simulink model "VirtualQuantumDotAgent"  (R2026a)
settings: Solver=FixedStepDiscrete  StartTime=0  StopTime=50e-9  FixedStep=1e-11
InitFcn:
  | qdEnsureWorkspace;
values from neighbouring files (symbols this model uses):
  QD_SAMPLE_TIME_S = 1.0e-11    (= 1e-11)    [initVirtualQuantumDotAgent.m]
  qdInput = qdDefaultInputs()    [initVirtualQuantumDotAgent.m]    (also in predictQDHybrid.m = defaults; predictQDWithError.m = defaults; qdDefaultInputs.m = struct(      'radius_nm', 3.0,      'temperature_K', 300.0, ; qdEnsureWorkspace.m = defaults)
undefined symbols (not defined in the file or in its folder): DiscIntNeverNeededParam
Description:
  | Virtual Quantum Dot Agent package model 1.2.0
settings Model: Creator=jyohtiprakash  LastModifiedBy=jyohtiprakash

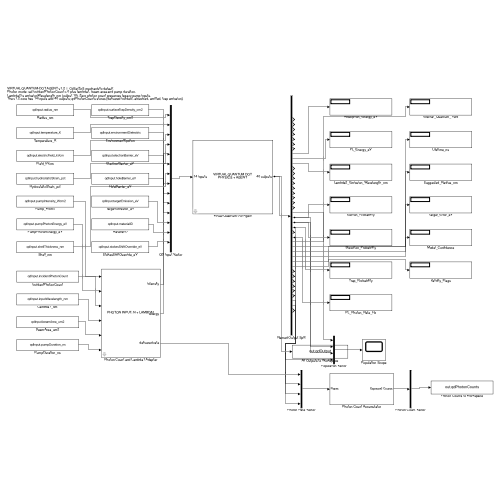
[thumbnail: Simulink's stored preview of the top-level diagram]
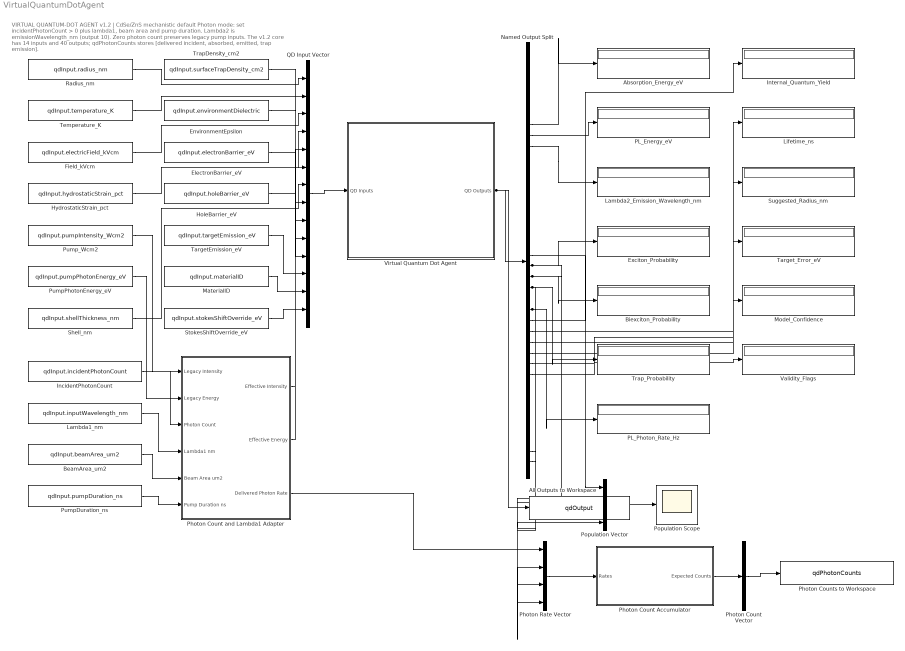
== system VirtualQuantumDotAgent ==
  note: VIRTUAL QUANTUM-DOT AGENT v1.2  |  CdSe/ZnS mechanistic default
      | Photon mode: set incidentPhotonCount > 0 plus lambda1, beam area and pump duration.
      | Lambda2 is emissionWavelength_nm (output 10). Zero photon count preserves legacy pump inputs.
      | The v1.2 core has 14 inputs and 40 outputs; qdPhotonCounts stores [delivered incident, absorbed, emitted, trap emission].
  Absorption_Energy_eV : Display
  All Outputs to Workspace : ToWorkspace  VariableName=qdOutput  SaveFormat=Structure With Time  SampleTime=-1
  BeamArea_um2 : Constant  Value=qdInput.beamArea_um2  SampleTime=QD_SAMPLE_TIME_S
  Biexciton_Probability : Display
  ElectronBarrier_eV : Constant  Value=qdInput.electronBarrier_eV  SampleTime=QD_SAMPLE_TIME_S
  EnvironmentEpsilon : Constant  Value=qdInput.environmentDielectric  SampleTime=QD_SAMPLE_TIME_S
  Exciton_Probability : Display
  Field_kVcm : Constant  Value=qdInput.electricField_kVcm  SampleTime=QD_SAMPLE_TIME_S
  HoleBarrier_eV : Constant  Value=qdInput.holeBarrier_eV  SampleTime=QD_SAMPLE_TIME_S
  HydrostaticStrain_pct : Constant  Value=qdInput.hydrostaticStrain_pct  SampleTime=QD_SAMPLE_TIME_S
  IncidentPhotonCount : Constant  Value=qdInput.incidentPhotonCount  SampleTime=QD_SAMPLE_TIME_S
  Internal_Quantum_Yield : Display
  Lambda1_nm : Constant  Value=qdInput.inputWavelength_nm  SampleTime=QD_SAMPLE_TIME_S
  Lambda2_Emission_Wavelength_nm : Display
  Lifetime_ns : Display
  MaterialID : Constant  Value=qdInput.materialID  SampleTime=QD_SAMPLE_TIME_S
  Model_Confidence : Display
  Named Output Split : Demux  Outputs=40
  PL_Energy_eV : Display
  PL_Photon_Rate_Hz : Display
  Photon Count Accumulator : Subsystem
  Photon Count Vector : Mux  Inputs=1
  Photon Count and Lambda1 Adapter : Subsystem
      mask help: Backward-compatible photon count and wavelength adapter for the 14-input quantum-dot core.
      mask Display:
      | disp('PHOTON INPUT: N + LAMBDA1');
      | port_label('output',1,'intensity');
      | port_label('output',2,'energy');
      | port_label('output',3,'delivered rate');
  Photon Counts to Workspace : ToWorkspace  VariableName=qdPhotonCounts  SaveFormat=Structure With Time  SampleTime=-1
  Photon Rate Vector : Mux
  Population Scope : Scope
  Population Vector : Mux
  PumpDuration_ns : Constant  Value=qdInput.pumpDuration_ns  SampleTime=QD_SAMPLE_TIME_S
  PumpPhotonEnergy_eV : Constant  Value=qdInput.pumpPhotonEnergy_eV  SampleTime=QD_SAMPLE_TIME_S
  Pump_Wcm2 : Constant  Value=qdInput.pumpIntensity_Wcm2  SampleTime=QD_SAMPLE_TIME_S
  QD Input Vector : Mux  Inputs=14
  Radius_nm : Constant  Value=qdInput.radius_nm  SampleTime=QD_SAMPLE_TIME_S
  Shell_nm : Constant  Value=qdInput.shellThickness_nm  SampleTime=QD_SAMPLE_TIME_S
  StokesShiftOverride_eV : Constant  Value=qdInput.stokesShiftOverride_eV  SampleTime=QD_SAMPLE_TIME_S
  Suggested_Radius_nm : Display
  TargetEmission_eV : Constant  Value=qdInput.targetEmission_eV  SampleTime=QD_SAMPLE_TIME_S
  Target_Error_eV : Display
  Temperature_K : Constant  Value=qdInput.temperature_K  SampleTime=QD_SAMPLE_TIME_S
  TrapDensity_cm2 : Constant  Value=qdInput.surfaceTrapDensity_cm2  SampleTime=QD_SAMPLE_TIME_S
  Trap_Probability : Display
  Validity_Flags : Display
  Virtual Quantum Dot Agent : Subsystem
      mask help: Effective-mass quantum-dot digital twin with population dynamics and inverse radius recommendation.
      mask Display:
      | disp('VIRTUAL QUANTUM DOT\nPHYSICS + AGENT');
      | port_label('input',1,'14 inputs');
      | port_label('output',1,'40 outputs');
  wires:
  Pump_Wcm2/1 -> Photon Count and Lambda1 Adapter/1(Legacy Intensity)
  PumpPhotonEnergy_eV/1 -> Photon Count and Lambda1 Adapter/2(Legacy Energy)
  IncidentPhotonCount/1 -> Photon Count and Lambda1 Adapter/3(Photon Count)
  Lambda1_nm/1 -> Photon Count and Lambda1 Adapter/4(Lambda1 nm)
  BeamArea_um2/1 -> Photon Count and Lambda1 Adapter/5(Beam Area um2)
  PumpDuration_ns/1 -> Photon Count and Lambda1 Adapter/6(Pump Duration ns)
  Radius_nm/1 -> QD Input Vector/1
  Temperature_K/1 -> QD Input Vector/2
  Field_kVcm/1 -> QD Input Vector/3
  HydrostaticStrain_pct/1 -> QD Input Vector/4
  Shell_nm/1 -> QD Input Vector/7
  TrapDensity_cm2/1 -> QD Input Vector/8
  EnvironmentEpsilon/1 -> QD Input Vector/9
  ElectronBarrier_eV/1 -> QD Input Vector/10
  HoleBarrier_eV/1 -> QD Input Vector/11
  TargetEmission_eV/1 -> QD Input Vector/12
  MaterialID/1 -> QD Input Vector/13
  StokesShiftOverride_eV/1 -> QD Input Vector/14
  Photon Count and Lambda1 Adapter/1(Effective Intensity) -> QD Input Vector/5
  Photon Count and Lambda1 Adapter/2(Effective Energy) -> QD Input Vector/6
  QD Input Vector/1 -> Virtual Quantum Dot Agent/1(QD Inputs)
  Virtual Quantum Dot Agent/1(QD Outputs) -> Named Output Split/1, All Outputs to Workspace/1
  Named Output Split/8 -> Absorption_Energy_eV/1
  Named Output Split/9 -> PL_Energy_eV/1
  Named Output Split/10 -> Lambda2_Emission_Wavelength_nm/1
  Named Output Split/21 -> Exciton_Probability/1, Population Vector/2
  Named Output Split/22 -> Biexciton_Probability/1, Population Vector/3
  Named Output Split/23 -> Trap_Probability/1, Population Vector/4
  Named Output Split/25 -> PL_Photon_Rate_Hz/1, Photon Rate Vector/3
  Named Output Split/26 -> Internal_Quantum_Yield/1
  Named Output Split/27 -> Lifetime_ns/1
  Named Output Split/28 -> Suggested_Radius_nm/1
  Named Output Split/29 -> Target_Error_eV/1
  Named Output Split/30 -> Model_Confidence/1
  Named Output Split/31 -> Validity_Flags/1
  Named Output Split/20 -> Population Vector/1
  Population Vector/1 -> Population Scope/1
  Photon Count and Lambda1 Adapter/3(Delivered Photon Rate) -> Photon Rate Vector/1
  Named Output Split/38 -> Photon Rate Vector/2
  Named Output Split/39 -> Photon Rate Vector/4
  Photon Rate Vector/1 -> Photon Count Accumulator/1(Rates)
  Photon Count Accumulator/1(Expected Counts) -> Photon Count Vector/1
  Photon Count Vector/1 -> Photon Counts to Workspace/1

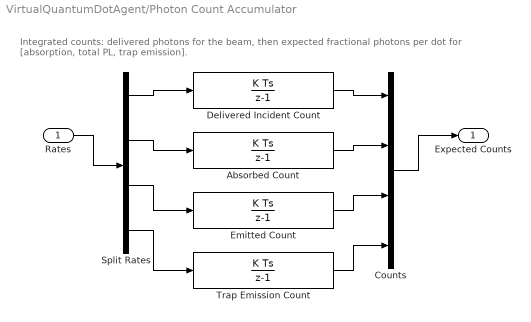
== system VirtualQuantumDotAgent/Photon Count Accumulator ==
  note: Integrated counts: delivered photons for the beam, then expected fractional photons per dot for [absorption, total PL, trap emission].
  Rates : Inport
  Absorbed Count : DiscreteIntegrator  gainval=1  SampleTime=QD_SAMPLE_TIME_S  ICPrevOutput=DiscIntNeverNeededParam  ICPrevScaledInput=DiscIntNeverNeededParam
  Counts : Mux
  Delivered Incident Count : DiscreteIntegrator  gainval=1  SampleTime=QD_SAMPLE_TIME_S  ICPrevOutput=DiscIntNeverNeededParam  ICPrevScaledInput=DiscIntNeverNeededParam
  Emitted Count : DiscreteIntegrator  gainval=1  SampleTime=QD_SAMPLE_TIME_S  ICPrevOutput=DiscIntNeverNeededParam  ICPrevScaledInput=DiscIntNeverNeededParam
  Split Rates : Demux
  Trap Emission Count : DiscreteIntegrator  gainval=1  SampleTime=QD_SAMPLE_TIME_S  ICPrevOutput=DiscIntNeverNeededParam  ICPrevScaledInput=DiscIntNeverNeededParam
  Expected Counts : Outport
  wires:
  Rates/1 -> Split Rates/1
  Split Rates/1 -> Delivered Incident Count/1
  Split Rates/2 -> Absorbed Count/1
  Split Rates/3 -> Emitted Count/1
  Split Rates/4 -> Trap Emission Count/1
  Delivered Incident Count/1 -> Counts/1
  Absorbed Count/1 -> Counts/2
  Emitted Count/1 -> Counts/3
  Trap Emission Count/1 -> Counts/4
  Counts/1 -> Expected Counts/1

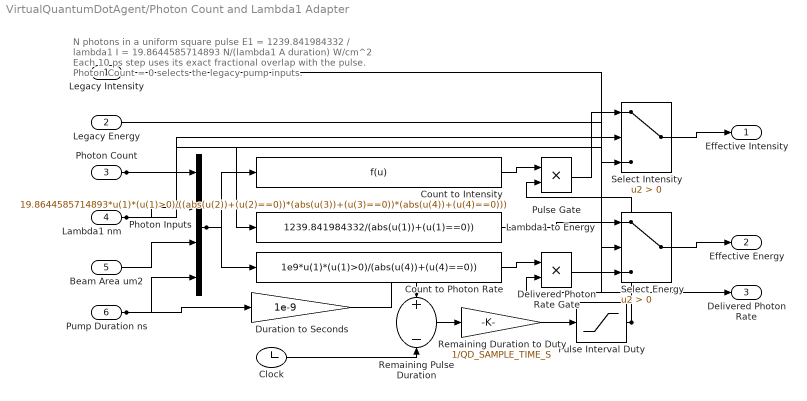
== system VirtualQuantumDotAgent/Photon Count and Lambda1 Adapter ==
  note: N photons in a uniform square pulse
      | E1 = 1239.841984332 / lambda1
      | I = 19.8644585714893 N/(lambda1 A duration) W/cm^2
      | Each 10 ps step uses its exact fractional overlap with the pulse.
      | Photon Count = 0 selects the legacy pump inputs.
  Legacy Intensity : Inport
  Legacy Energy : Inport  Port=2
  Photon Count : Inport  Port=3
  Lambda1 nm : Inport  Port=4
  Beam Area um2 : Inport  Port=5
  Pump Duration ns : Inport  Port=6
  Clock : Clock
  Count to Intensity : Fcn  Expr=19.8644585714893*u(1)*(u(1)>0)/((abs(u(2))+(u(2)==0))*(abs(u(3))+(u(3)==0))*(abs(u(4))+(u(4)==0)))
  Count to Photon Rate : Fcn  Expr=1e9*u(1)*(u(1)>0)/(abs(u(4))+(u(4)==0))
  Delivered Photon Rate Gate : Product  Inputs=**
  Duration to Seconds : Gain  Gain=1e-9
  Lambda1 to Energy : Fcn  Expr=1239.841984332/(abs(u(1))+(u(1)==0))
  Photon Inputs : Mux
  Pulse Gate : Product  Inputs=**
  Pulse Interval Duty : Saturate  UpperLimit=1  LowerLimit=0
  Remaining Duration to Duty : Gain  Gain=1/QD_SAMPLE_TIME_S
  Remaining Pulse Duration : Sum  Inputs=+-
  Select Energy : Switch  Criteria=u2 > Threshold  SaturateOnIntegerOverflow=off  InputSameDT=off
  Select Intensity : Switch  Criteria=u2 > Threshold  SaturateOnIntegerOverflow=off  InputSameDT=off
  Effective Intensity : Outport
  Effective Energy : Outport  Port=2
  Delivered Photon Rate : Outport  Port=3
  wires:
  Photon Count/1 -> Photon Inputs/1, Select Intensity/2, Select Energy/2
  Lambda1 nm/1 -> Photon Inputs/2, Lambda1 to Energy/1
  Beam Area um2/1 -> Photon Inputs/3
  Pump Duration ns/1 -> Photon Inputs/4, Duration to Seconds/1
  Photon Inputs/1 -> Count to Intensity/1, Count to Photon Rate/1
  Duration to Seconds/1 -> Remaining Pulse Duration/1
  Clock/1 -> Remaining Pulse Duration/2
  Remaining Pulse Duration/1 -> Remaining Duration to Duty/1
  Remaining Duration to Duty/1 -> Pulse Interval Duty/1
  Count to Intensity/1 -> Pulse Gate/1
  Pulse Interval Duty/1 -> Pulse Gate/2, Delivered Photon Rate Gate/2
  Count to Photon Rate/1 -> Delivered Photon Rate Gate/1
  Pulse Gate/1 -> Select Intensity/1
  Legacy Intensity/1 -> Select Intensity/3
  Lambda1 to Energy/1 -> Select Energy/1
  Legacy Energy/1 -> Select Energy/3
  Select Intensity/1 -> Effective Intensity/1
  Select Energy/1 -> Effective Energy/1
  Delivered Photon Rate Gate/1 -> Delivered Photon Rate/1

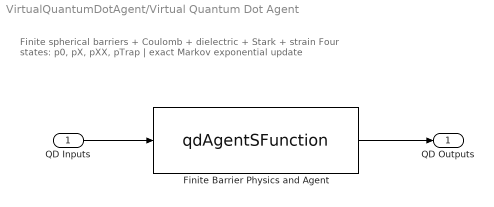
== system VirtualQuantumDotAgent/Virtual Quantum Dot Agent ==
  note: Finite spherical barriers + Coulomb + dielectric + Stark + strain
      | Four states: p0, pX, pXX, pTrap | exact Markov exponential update
  QD Inputs : Inport  PortDimensions=14
  Finite Barrier Physics and Agent : M-S-Function  FunctionName=qdAgentSFunction
  QD Outputs : Outport
  wires:
  QD Inputs/1 -> Finite Barrier Physics and Agent/1
  Finite Barrier Physics and Agent/1 -> QD Outputs/1
